simulink model "motor"  (R2024b)
settings: Solver=VariableStepAuto  StartTime=0.0  StopTime=0.3  RelTol=1e-3
values from neighbouring files (symbols this model uses):
  A = [-Ra/La -K/La; K/J 0]    [lab.m]
  B = [1/La  0; 0 -1/J]    [lab.m]
  C = [1 0; 0 1]    [lab.m]
  D = [0 0; 0 0]    [lab.m]
  den11 = cell2mat(den11)    [lab.m]
  den12 = cell2mat(den12)    [lab.m]
  den21 = cell2mat(den21)    [lab.m]
  den22 = cell2mat(den22)    [lab.m]
  num11 = cell2mat(num11)    [lab.m]
  num12 = cell2mat(num12)    [lab.m]
  num21 = cell2mat(num21)    [lab.m]
  num22 = cell2mat(num22)    [lab.m]
settings Model: Creator=rober  LastModifiedBy=rober

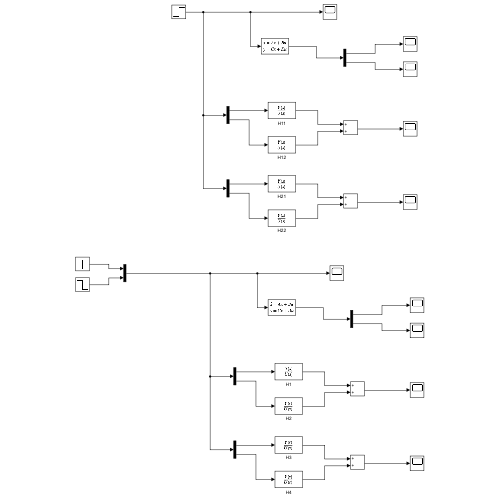
[thumbnail: Simulink's stored preview of the top-level diagram]
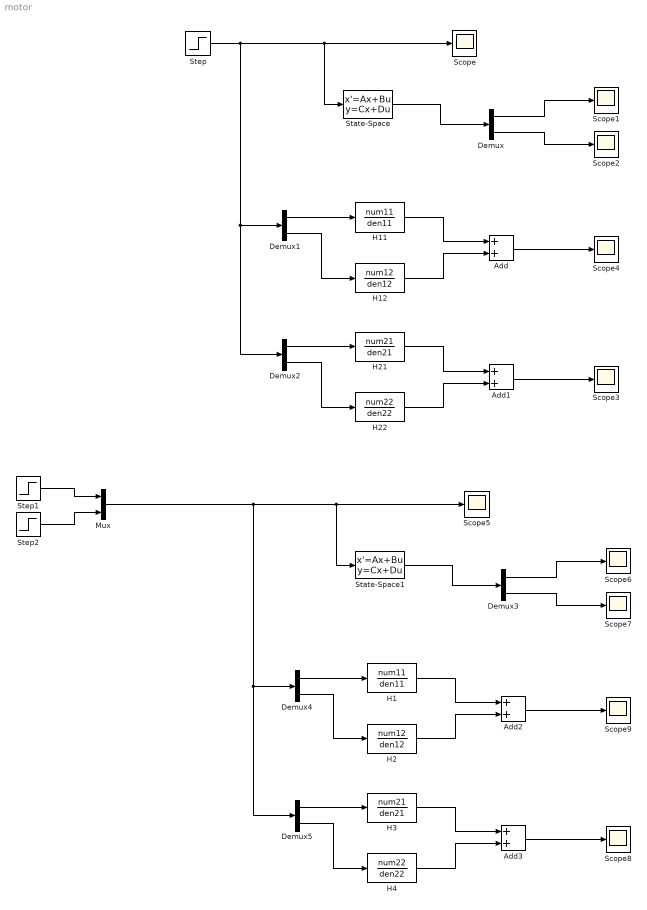
== system motor ==
  Add{,1..3} (4 alike) : Sum
  Demux{,1..5} (6 alike) : Demux  Outputs=2
  H1 : TransferFcn  Numerator=num11  Denominator=den11
  H11 : TransferFcn  Numerator=num11  Denominator=den11
  H12 : TransferFcn  Numerator=num12  Denominator=den12
  H2 : TransferFcn  Numerator=num12  Denominator=den12
  H21 : TransferFcn  Numerator=num21  Denominator=den21
  H22 : TransferFcn  Numerator=num22  Denominator=den22
  H3 : TransferFcn  Numerator=num21  Denominator=den21
  H4 : TransferFcn  Numerator=num22  Denominator=den22
  Mux : Mux  Inputs=2
  Scope{,1..9} (10 alike) : Scope
  State-Space : StateSpace  A=A  B=B  C=C  D=D  InitialCondition=0
  State-Space1 : StateSpace  A=A  B=B  C=C  D=D  InitialCondition=0
  Step : Step  Time=0  After=[24 0.04]  SampleTime=0
  Step1 : Step  Time=0.1  Before=24  After=0  SampleTime=0
  Step2 : Step  Time=0.2  Before=0.04  After=-0.21  SampleTime=0
  wires:
  Step/1 -> Demux2/1, Demux1/1, State-Space/1, Scope/1
  State-Space/1 -> Demux/1
  Demux/1 -> Scope1/1
  Demux/2 -> Scope2/1
  H12/1 -> Add/2
  Demux1/2 -> H12/1
  Demux1/1 -> H11/1
  H11/1 -> Add/1
  Demux2/1 -> H21/1
  Demux2/2 -> H22/1
  Add/1 -> Scope4/1
  H21/1 -> Add1/1
  Add1/1 -> Scope3/1
  H22/1 -> Add1/2
  Demux5/1 -> H3/1
  H1/1 -> Add2/1
  Add2/1 -> Scope9/1
  Demux5/2 -> H4/1
  H2/1 -> Add2/2
  H3/1 -> Add3/1
  H4/1 -> Add3/2
  State-Space1/1 -> Demux3/1
  Demux3/1 -> Scope6/1
  Demux3/2 -> Scope7/1
  Demux4/2 -> H2/1
  Mux/1 -> Demux5/1, Demux4/1, State-Space1/1, Scope5/1
  Add3/1 -> Scope8/1
  Demux4/1 -> H1/1
  Step1/1 -> Mux/1
  Step2/1 -> Mux/2
